simulink model "QPSK_over_fading_channels"  (R2024a)
settings: Solver=VariableStepAuto  StartTime=0.0  StopTime=10.0  RelTol=1e-3
undefined symbols (not defined in the file): doppler
libraries: commchan3 x2, commrandsrc3 x1, commdigbbndpm3 x1
settings Model: Creator=Anusnekhaa Narendran  LastModifiedBy=Anusnekhaa Narendran

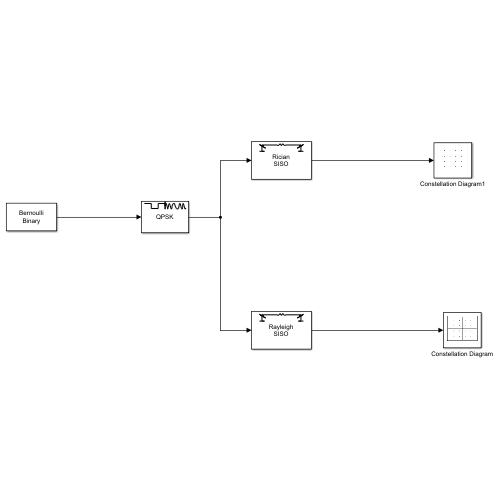
[thumbnail: Simulink's stored preview of the top-level diagram]
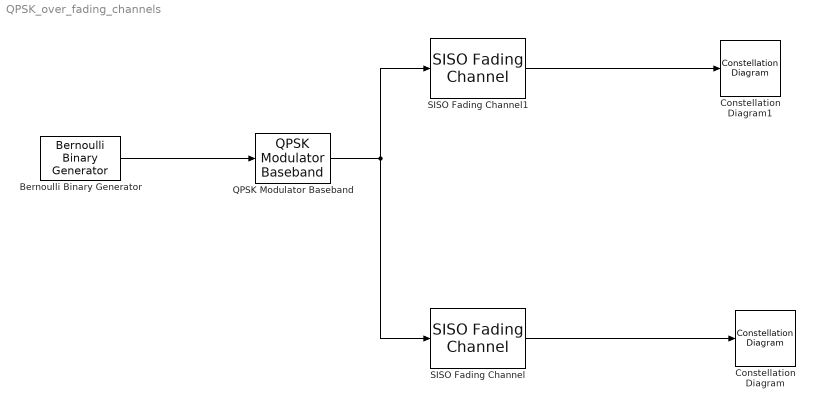
== system QPSK_over_fading_channels ==
  Bernoulli Binary Generator : commrandsrc3/Bernoulli Binary Generator  ProbabilityOfZero=0.5  SeedSource=Auto  Seed=0  SampleTime=1/50000  SamplesPerFrame=100  OutputDataType=boolean  SimulateUsing=Interpreted execution
  Constellation Diagram : ConstellationDiagram  WindowPosition=[382.000000,84.000000,600.000000,600.000000,]  ScopeFrameLocation=window  XLimits=[-5.8,5.8]  YLimits=[-2.75,2.75]  ShowGrid=off
  Constellation Diagram1 : ConstellationDiagram  WindowPosition=[382.000000,84.000000,600.000000,600.000000,]  ScopeFrameLocation=window
  QPSK Modulator Baseband : commdigbbndpm3/QPSK Modulator Baseband  InType=Bit  Enc=Gray  Ph=pi/4  outDtype=double  outWordLen=16  outUDDataType=sfix(16)  outFracLenMode=Best precision  outFracLen=15  outDataTypeStr=double  outLastDataTypeStr=double
  SISO Fading Channel : commchan3/SISO Fading Channel  InheritSampleRate=on  SampleRate=1  PathDelays=[5e-5 15e-5 20e-5]  AveragePathGains=[0 -3 -9]  NormalizePathGains=on  FadingDistribution=Rayleigh  KFactor=3  DirectPathDopplerShift=0  DirectPathInitialPhase=0  MaximumDopplerShift=0.00001  DopplerSpectrum=doppler('Jakes')  RandomStream=mt19937ar with seed  Seed=73  PathGainsOutputPort=off  ChannelFilterDelayOutputPort=off  SimulateUsing=Interpreted execution  Visualization=Impulse response  PathsForDopplerDisplay=1  SamplesToDisplay=25%
  SISO Fading Channel1 : commchan3/SISO Fading Channel  InheritSampleRate=on  SampleRate=1  PathDelays=[0 15e-5 20e-5]  AveragePathGains=[0 -3 -9]  NormalizePathGains=on  FadingDistribution=Rician  KFactor=1  DirectPathDopplerShift=0.000001  DirectPathInitialPhase=0  MaximumDopplerShift=1  DopplerSpectrum=doppler('Jakes')  RandomStream=mt19937ar with seed  Seed=73  PathGainsOutputPort=off  ChannelFilterDelayOutputPort=off  SimulateUsing=Interpreted execution  Visualization=Frequency response  PathsForDopplerDisplay=1  SamplesToDisplay=50%
  wires:
  Bernoulli Binary Generator/1 -> QPSK Modulator Baseband/1
  QPSK Modulator Baseband/1 -> SISO Fading Channel1/1, SISO Fading Channel/1
  SISO Fading Channel1/1 -> Constellation Diagram1/1
  SISO Fading Channel/1 -> Constellation Diagram/1
